simulink library "Lib_Piccolo"  (R2018b)
settings: Solver=VariableStepAuto  StartTime=0.0  StopTime=10.0  RelTol=1e-3
values from neighbouring files (symbols this model uses):
  AccelErrInt2Brakes = 0.15    [SimulationControlConfig16P.m]    (also in SimulationControlConfig16P_LEGACY.m; SimulationControlConfigTAILLESS.m = 0.2; SimulationControlConfigUTAIL.m = 0.2)
  AileronMax = 25    [SimulationControlConfig16P.m]    (also in SimulationControlConfig16P_LEGACY.m; SimulationControlConfigTAILLESS.m; SimulationControlConfigUTAIL.m)
  AileronPower = 0.00268    [SimulationControlConfig16P.m]    (also in SimulationControlConfig16P_LEGACY.m; SimulationControlConfigTAILLESS.m; SimulationControlConfigUTAIL.m)
  AileronSurfaceMax = 45    [SimulationControlConfig16P.m]    (also in SimulationControlConfig16P_LEGACY.m)
  AileronTrim = 0    [SimulationControlConfig16P.m]    (also in SimulationControlConfig16P_LEGACY.m; SimulationControlConfigTAILLESS.m; SimulationControlConfigUTAIL.m)
  Alt = 1000 + TerrainHeight    [SimulationStateConfig.m]
  AltCruise_m = testPlans(testIndx).terrainElevation * 0.3048 + 200    [SimulationControlConfig16P.m]    (also in SimulationControlConfigTAILLESS.m = 1083; SimulationControlConfigUTAIL.m = testPlans(testIndx).terrainElevation * 0.3048 + 152)
  AltitudeRate2PitchCmdIntegratorInit = 0.1    [SimulationControlPre.m]
  AltMax = 10000    [SimulationControlConfig16P.m]    (also in SimulationControlConfig16P_LEGACY.m; SimulationControlConfigTAILLESS.m; SimulationControlConfigUTAIL.m)
  AltMaxAccel = 1.25    [SimulationControlConfig16P.m]    (also in SimulationControlConfig16P_LEGACY.m = 0.9; SimulationControlConfigTAILLESS.m = 1.7; SimulationControlConfigUTAIL.m = 2)
  AltMin = 0    [SimulationControlConfig16P.m]    (also in SimulationControlConfig16P_LEGACY.m; SimulationControlConfigTAILLESS.m; SimulationControlConfigUTAIL.m)
  AltRateCmd2Pitch = 0.50    (= 0.5)    [SimulationControlConfig16P.m]    (also in SimulationControlConfig16P_LEGACY.m = 0.6; SimulationControlConfigTAILLESS.m = 0.2; SimulationControlConfigUTAIL.m = 0.3)
  AltRateError2Pitch = 0.40    (= 0.4)    [SimulationControlConfig16P.m]    (also in SimulationControlConfig16P_LEGACY.m; SimulationControlConfigTAILLESS.m = 0.55; SimulationControlConfigUTAIL.m = 0.55)
  AltRateErrorInt2Pitch = 0.50    (= 0.5)    [SimulationControlConfig16P.m]    (also in SimulationControlConfig16P_LEGACY.m = 0.45; SimulationControlConfigTAILLESS.m; SimulationControlConfigUTAIL.m = 0.75)
  AltRateLpfCutOff = 3    [SimulationControlConfig16P.m]    (also in SimulationControlConfig16P_LEGACY.m; SimulationControlConfigTAILLESS.m = 2; SimulationControlConfigUTAIL.m = 2)
  AutoNosegear2Rudder = 26    [SimulationControlConfig16P.m]    (also in SimulationControlConfig16P_LEGACY.m; SimulationControlConfigTAILLESS.m = 25.2; SimulationControlConfigUTAIL.m = 14)
  b = 5.54    [SimulationControlConfig16P.m]    (also in SimulationControlConfig16P_LEGACY.m; SimulationControlConfigTAILLESS.m = 2.37; SimulationControlConfigUTAIL.m = 2.37)
  Bank2AileronIntegratorInit = 0    [SimulationControlPre.m]
  BankMax_User = BankMax_User/180*pi    (= 0.523598775598)    [SimulationControlConfig16P.m]    (also in SimulationControlConfig16P_LEGACY.m; SimulationControlConfigTAILLESS.m = 0.610865238198; SimulationControlConfigUTAIL.m = 0.628318530718)
  baseLegFlaps = 20    [SimulationControlConfig16P.m]    (also in SimulationControlConfig16P_LEGACY.m = 0; SimulationControlConfigTAILLESS.m = 15; SimulationControlConfigUTAIL.m = 10)
  C = GeneticOpt.C    [SimulationCostFunction.m]
  c = Sw/b    (= 0.841696750903)    [SimulationControlConfig16P.m]    (also in SimulationControlConfig16P_LEGACY.m; SimulationControlConfigTAILLESS.m = 0.354008438819; SimulationControlConfigUTAIL.m = 0.354008438819)
  cell2WheelFactorMG = 5.98    [SimulationSensorConfig16P_LEGACY.m]
  cell2WheelFactorNG = 1    [SimulationSensorConfig16P_LEGACY.m]
  cellSatMaxMG = 15000    [SimulationSensorConfig16P.m]    (also in SimulationSensorConfig16P_LEGACY.m; SimulationSensorConfigTAILLESS7P.m; SimulationSensorConfigUTAIL7P.m)
  cellSatMaxNG = 1000    [SimulationSensorConfig16P.m]    (also in SimulationSensorConfig16P_LEGACY.m; SimulationSensorConfigTAILLESS7P.m; SimulationSensorConfigUTAIL7P.m)
  cellSatMinMG = -15000    [SimulationSensorConfig16P.m]    (also in SimulationSensorConfig16P_LEGACY.m; SimulationSensorConfigTAILLESS7P.m; SimulationSensorConfigUTAIL7P.m)
  cellSatMinNG = -1000    [SimulationSensorConfig16P.m]    (also in SimulationSensorConfig16P_LEGACY.m; SimulationSensorConfigTAILLESS7P.m; SimulationSensorConfigUTAIL7P.m)
  CL_Limit = CL_Max    (= 0.54)    [SimulationControlConfig16P.m]    (also in SimulationControlConfig16P_LEGACY.m; SimulationControlConfigTAILLESS.m; SimulationControlConfigUTAIL.m = 0.53)
  CL_Max = 0.54    [SimulationControlConfig16P.m]    (also in SimulationControlConfig16P_LEGACY.m; SimulationControlConfigTAILLESS.m; SimulationControlConfigUTAIL.m = 0.53)
  CL_Max_Nom = 0.465    [SimulationControlConfig16P.m]    (also in SimulationControlConfig16P_LEGACY.m; SimulationControlConfigTAILLESS.m = 0.39; SimulationControlConfigUTAIL.m)
  CL_Min = 0    [SimulationControlConfig16P.m]    (also in SimulationControlConfig16P_LEGACY.m; SimulationControlConfigTAILLESS.m; SimulationControlConfigUTAIL.m)
  ClimbMaxFraction = 0.35    [SimulationControlConfig16P.m]    (also in SimulationControlConfig16P_LEGACY.m = 0.24; SimulationControlConfigTAILLESS.m = 0.19; SimulationControlConfigUTAIL.m = 0.21)
  ClimboutMaxBank = 7.0    (= 7)    [SimulationControlConfig16P.m]    (also in SimulationControlConfig16P_LEGACY.m; SimulationControlConfigTAILLESS.m = 5; SimulationControlConfigUTAIL.m)
  ClimboutTimer = 7.0    (= 7)    [SimulationControlConfig16P.m]    (also in SimulationControlConfig16P_LEGACY.m; SimulationControlConfigTAILLESS.m; SimulationControlConfigUTAIL.m)
  dCl_per_dFlap = 0.005581818    [SimulationControlConfig16P.m]    (also in SimulationControlConfig16P_LEGACY.m = 0; SimulationControlConfigTAILLESS.m = 0; SimulationControlConfigUTAIL.m = 0)
  DecelerationCmd = 3.1    [SimulationControlConfig16P.m]    (also in SimulationControlConfig16P_LEGACY.m; SimulationControlConfigTAILLESS.m = 0.1; SimulationControlConfigUTAIL.m = 0.1)
  DeRotateLogicEndTimer = abs((NoseDownLimit_Deg-1)/DeRotateRamp_Dps)    [SimulationControlConfig16P.m]    (also in SimulationControlConfig16P_LEGACY.m; SimulationControlConfigTAILLESS.m; SimulationControlConfigUTAIL.m)
  DeRotateLogicHoldNoseUpTimer = 0.1    [SimulationControlConfig16P.m]    (also in SimulationControlConfig16P_LEGACY.m; SimulationControlConfigTAILLESS.m; SimulationControlConfigUTAIL.m)
  DeRotateLogicTimerTimeout = 2    [SimulationControlConfig16P.m]    (also in SimulationControlConfig16P_LEGACY.m; SimulationControlConfigTAILLESS.m; SimulationControlConfigUTAIL.m)
  DeRotateLowerCmdSaturation = 0    [SimulationControlConfig16P.m]    (also in SimulationControlConfig16P_LEGACY.m; SimulationControlConfigTAILLESS.m; SimulationControlConfigUTAIL.m)
  DeRotateRamp_Dps = 3    [SimulationControlConfig16P.m]    (also in SimulationControlConfig16P_LEGACY.m; SimulationControlConfigTAILLESS.m = 8; SimulationControlConfigUTAIL.m = 8)
  DeRotateUpperCmdSaturation = 7    [SimulationControlConfig16P.m]    (also in SimulationControlConfig16P_LEGACY.m; SimulationControlConfigTAILLESS.m; SimulationControlConfigUTAIL.m)
  DescentMaxFraction = 0.22    [SimulationControlConfig16P.m]    (also in SimulationControlConfig16P_LEGACY.m = 0.2; SimulationControlConfigTAILLESS.m = 0.17; SimulationControlConfigUTAIL.m = 0.17)
  DesktopSimTerrainOffset_m = 0.406    [SimulationAircraftConfig.m]
  downwindFlaps = 0    [SimulationControlConfig16P.m]    (also in SimulationControlConfig16P_LEGACY.m; SimulationControlConfigTAILLESS.m; SimulationControlConfigUTAIL.m)
  DP_init = 0.5*1.225*V_init^2    [SimulationControlConfig16P.m]    (also in SimulationControlConfig16P_LEGACY.m; SimulationControlConfigTAILLESS.m; SimulationControlConfigUTAIL.m)
  dscNoiseMG = 1    [SimulationSensorConfig16P_LEGACY.m]
  dscNoiseNG = 0.25    [SimulationSensorConfig16P_LEGACY.m]
  DSCnumBits = 24    [SimulationSensorConfig16P.m]    (also in SimulationSensorConfig16P_LEGACY.m; SimulationSensorConfigTAILLESS7P.m; SimulationSensorConfigUTAIL7P.m)
  DSCRangeMaxMG = 15000    [SimulationSensorConfig16P.m]    (also in SimulationSensorConfig16P_LEGACY.m; SimulationSensorConfigTAILLESS7P.m; SimulationSensorConfigUTAIL7P.m)
  DSCRangeMaxNG = 1000    [SimulationSensorConfig16P.m]    (also in SimulationSensorConfig16P_LEGACY.m; SimulationSensorConfigTAILLESS7P.m; SimulationSensorConfigUTAIL7P.m)
  DSCRangeMinMG = -15000    [SimulationSensorConfig16P.m]    (also in SimulationSensorConfig16P_LEGACY.m; SimulationSensorConfigTAILLESS7P.m; SimulationSensorConfigUTAIL7P.m)
  DSCRangeMinNG = -1000    [SimulationSensorConfig16P.m]    (also in SimulationSensorConfig16P_LEGACY.m; SimulationSensorConfigTAILLESS7P.m; SimulationSensorConfigUTAIL7P.m)
  dt = DLLSim.dt    [SimulationTimeStep.m]    (also in SimulationTrim.m = 0.02)
  EarlyTouchdownThreshold = 3.0    (= 3)    [SimulationControlConfig16P.m]    (also in SimulationControlConfig16P_LEGACY.m; SimulationControlConfigTAILLESS.m = 2.2; SimulationControlConfigUTAIL.m = 2.5)
  ElevatorDeflectionRate = 15    [SimulationControlConfig16P.m]    (also in SimulationControlConfig16P_LEGACY.m = 12; SimulationControlConfigTAILLESS.m = 10; SimulationControlConfigUTAIL.m = 12)
  ElevatorMax = 25    [SimulationControlConfig16P.m]    (also in SimulationControlConfig16P_LEGACY.m; SimulationControlConfigTAILLESS.m; SimulationControlConfigUTAIL.m)
  ElevatorPower = -0.002209    [SimulationControlConfig16P.m]    (also in SimulationControlConfig16P_LEGACY.m; SimulationControlConfigTAILLESS.m = -0.002956; SimulationControlConfigUTAIL.m = -0.00205983)
  ElevatorTrim = -3.5    [SimulationControlConfig16P.m]    (also in SimulationControlConfig16P_LEGACY.m; SimulationControlConfigTAILLESS.m = -6; SimulationControlConfigUTAIL.m = -8)
  elevonBias = 0    [SimulationControlConfig16P.m]    (also in SimulationControlConfig16P_LEGACY.m; SimulationControlConfigTAILLESS.m; SimulationControlConfigUTAIL.m)
  Enable_TAS_Protection = 0    [SimulationControlConfig16P.m]    (also in SimulationControlConfig16P_LEGACY.m; SimulationControlConfigTAILLESS.m; SimulationControlConfigUTAIL.m)
  EnableCrossTrackAbort = 1    [SimulationControlConfig16P.m]    (also in SimulationControlConfigTAILLESS.m; SimulationControlConfigUTAIL.m)
  EnergyBandwidth = 0.02    [SimulationControlConfig16P.m]    (also in SimulationControlConfig16P_LEGACY.m; SimulationControlConfigTAILLESS.m = 0.06; SimulationControlConfigUTAIL.m = 0.06)
  EngineLhFuelCut = 0    [SimulationAircraftConfig.m]
  EngineRhFuelCut = 0    [SimulationAircraftConfig.m]
  FastThrottleRate = 0.075    [SimulationControlConfig16P.m]    (also in SimulationControlConfig16P_LEGACY.m = 0.05; SimulationControlConfigTAILLESS.m = 0.1; SimulationControlConfigUTAIL.m = 0.1)
  FilterWarmUpTime = 2    [SimulationSensorConfig16P.m]    (also in SimulationSensorConfig16P_LEGACY.m; SimulationSensorConfigTAILLESS7P.m; SimulationSensorConfigUTAIL7P.m)
  finalApproachFlaps = 20    [SimulationControlConfig16P.m]    (also in SimulationControlConfig16P_LEGACY.m = 0; SimulationControlConfigTAILLESS.m = 22; SimulationControlConfigUTAIL.m = 10)
  FinalDescentSlope_Deg = testPlans(testIndx).descentSlope    [SimulationControlConfig16P.m]    (also in SimulationControlConfig16P_LEGACY.m; SimulationControlConfigTAILLESS.m; SimulationControlConfigUTAIL.m)
  flapMax = 0    [SimulationControlConfig16P.m]    (also in SimulationControlConfig16P_LEGACY.m; SimulationControlConfigTAILLESS.m; SimulationControlConfigUTAIL.m)
  flapRate = 7.5    [SimulationControlConfig16P.m]    (also in SimulationControlConfig16P_LEGACY.m; SimulationControlConfigTAILLESS.m = 6.6; SimulationControlConfigUTAIL.m)
  FlareHeight = 5    [SimulationControlConfig16P.m]    (also in SimulationControlConfig16P_LEGACY.m = 4.8; SimulationControlConfigTAILLESS.m = 2.5; SimulationControlConfigUTAIL.m = 2)
  FlareVerticalRate_mps = -0.4    [SimulationControlConfig16P.m]    (also in SimulationControlConfig16P_LEGACY.m = -0.5; SimulationControlConfigTAILLESS.m = -0.15; SimulationControlConfigUTAIL.m = -0.15)
  Fp_Aileron = 0.55*2*pi*RollRateLpfCutoff*dt    [SimulationControlConfig16P.m]    (also in SimulationControlConfig16P_LEGACY.m; SimulationControlConfigTAILLESS.m; SimulationControlConfigUTAIL.m)
  Fp_Alt = 0.55*AltBandwidth    (= 0.099)    [SimulationControlConfig16P.m]    (also in SimulationControlConfig16P_LEGACY.m; SimulationControlConfigTAILLESS.m = 0.587477826221; SimulationControlConfigUTAIL.m = 0.69115038379)
  Fp_AltRate = 0.55*2*pi*AltRateLpfCutOff*dt    [SimulationControlConfig16P.m]    (also in SimulationControlConfig16P_LEGACY.m; SimulationControlConfigTAILLESS.m; SimulationControlConfigUTAIL.m)
  Fp_Elevator = 0.55*2*pi*PitchRateLpfCutoff*dt    [SimulationControlConfig16P.m]    (also in SimulationControlConfig16P_LEGACY.m; SimulationControlConfigTAILLESS.m; SimulationControlConfigUTAIL.m)
  Fp_Energy = 0.55*2*pi*EnergyBandwidth    (= 0.069115038379)    [SimulationControlConfig16P.m]    (also in SimulationControlConfig16P_LEGACY.m; SimulationControlConfigTAILLESS.m = 0.207345115137; SimulationControlConfigUTAIL.m = 0.207345115137)
  Fp_Energy2 = 0.55*2*pi*EnergyBandwidth*dt    [SimulationControlConfig16P.m]    (also in SimulationControlConfig16P_LEGACY.m; SimulationControlConfigTAILLESS.m; SimulationControlConfigUTAIL.m)
  Fp_Pitch = 0.55*2*pi*PitchBandwidth    (= 2.76460153516)    [SimulationControlConfig16P.m]    (also in SimulationControlConfig16P_LEGACY.m = 3.11017672705; SimulationControlConfigTAILLESS.m = 3.80132711084; SimulationControlConfigUTAIL.m = 2.41902634326)
  Fp_Pitch_2 = 0.55*2*pi*PitchBandwidth*dt    [SimulationControlConfig16P.m]    (also in SimulationControlConfig16P_LEGACY.m; SimulationControlConfigTAILLESS.m; SimulationControlConfigUTAIL.m)
  Fp_Roll = RollBandwidth^2    (= 1)    [SimulationControlConfig16P.m]    (also in SimulationControlConfig16P_LEGACY.m = 1.44; SimulationControlConfigTAILLESS.m; SimulationControlConfigUTAIL.m)
  Fp_Rudder = 0.55*2*pi*YawRateLpfCutoff*dt    [SimulationControlConfig16P.m]    (also in SimulationControlConfig16P_LEGACY.m; SimulationControlConfigTAILLESS.m; SimulationControlConfigUTAIL.m)
  Fp_TAS = 0.55*2*pi*TASBandwidth    (= 0.103672557568)    [SimulationControlConfig16P.m]    (also in SimulationControlConfig16P_LEGACY.m; SimulationControlConfigTAILLESS.m = 0.172787595947; SimulationControlConfigUTAIL.m = 0.172787595947)
  Fp_TAS_Filter = 2*pi*TasLpfCutoff*dt    [SimulationControlConfig16P.m]    (also in SimulationControlConfig16P_LEGACY.m; SimulationControlConfigTAILLESS.m; SimulationControlConfigUTAIL.m)
  Fp_Turn = 0.55*2*pi*TurnErrLPFcutoff    (= 0.0345575191895)    [SimulationControlConfig16P.m]    (also in SimulationControlConfig16P_LEGACY.m; SimulationControlConfigTAILLESS.m = 0.172787595947; SimulationControlConfigUTAIL.m = 0.172787595947)
  Fp_TurnDerr = 0.55*2*pi*TurnDerivativeLPFcutoff    (= 0.0345575191895)    [SimulationControlConfig16P.m]    (also in SimulationControlConfig16P_LEGACY.m; SimulationControlConfigTAILLESS.m = 0.172787595947; SimulationControlConfigUTAIL.m = 0.172787595947)
  FTV = 3    [SimulationAircraftConfig.m]
  ftvStaticPositionError = 1/1.18    (= 0.847457627119)    [SimulationSensorConfig16P.m]    (also in SimulationSensorConfig16P_LEGACY.m; SimulationSensorConfigTAILLESS7P.m = 1; SimulationSensorConfigUTAIL7P.m = 1)
  g = 9.81    [SimulationStateConfig.m]
  GustSpd_Kts = testPlans(testIndx).gustSpd    [SimulationStateConfig.m]
  GustTriggerVal = testPlans(testIndx).gustTriggerVal    [SimulationStateConfig.m]
  HeadingErr2TurnRate = 0.5    [SimulationControlConfig16P.m]    (also in SimulationControlConfig16P_LEGACY.m; SimulationControlConfigTAILLESS.m; SimulationControlConfigUTAIL.m)
  HeadingErrDer2TurnRate = 0.3    [SimulationControlConfig16P.m]    (also in SimulationControlConfig16P_LEGACY.m; SimulationControlConfigTAILLESS.m; SimulationControlConfigUTAIL.m)
  IASbounce = IASstall*0.8    [SimulationControlPre.m]
  IAScruiseCMD = sqrt(2*m*9.81/(1.225*Sw*CL_cruise))    [SimulationControlConfig16P.m]    (also in SimulationControlConfig16P_LEGACY.m; SimulationControlConfigTAILLESS.m; SimulationControlConfigUTAIL.m)
  IASfinalCMD = 1.12 * IASmin    [SimulationControlConfig16P.m]    (also in SimulationControlConfig16P_LEGACY.m = 1.10 * IASmin; SimulationControlConfigTAILLESS.m = 1.10 * IASmin; SimulationControlConfigUTAIL.m = 1.15 * IASmin)
  IASflareCMD = IASstall    [SimulationControlConfig16P.m]    (also in SimulationControlConfig16P_LEGACY.m; SimulationControlConfigTAILLESS.m; SimulationControlConfigUTAIL.m)
  IASmax = 64    [SimulationControlConfig16P.m]    (also in SimulationControlConfig16P_LEGACY.m = 46; SimulationControlConfigTAILLESS.m = 38.58; SimulationControlConfigUTAIL.m = 35)
  IASmin = sqrt(2*m*9.81/(1.225*Sw*0.9*CL_Max_Nom))    [SimulationControlConfig16P.m]    (also in SimulationControlConfig16P_LEGACY.m; SimulationControlConfigTAILLESS.m; SimulationControlConfigUTAIL.m)
  IASshortCMD = IASstall    [SimulationControlConfig16P.m]    (also in SimulationControlConfig16P_LEGACY.m; SimulationControlConfigTAILLESS.m; SimulationControlConfigUTAIL.m)
  IASstall = sqrt(2*m*9.81/(1.225*Sw*CL_Max))    [SimulationControlConfig16P.m]    (also in SimulationControlConfig16P_LEGACY.m; SimulationControlConfigTAILLESS.m; SimulationControlConfigUTAIL.m)
  inFlight = 1    [SimulationControlConfig16P.m]    (also in SimulationControlConfigTAILLESS.m; SimulationControlConfigUTAIL.m)
  JetCatOffset = 5    [SimulationControlConfig16P.m]    (also in SimulationControlConfig16P_LEGACY.m)
  LaunchRollingElevator = -1.5    [SimulationControlConfig16P.m]    (also in SimulationControlConfig16P_LEGACY.m; SimulationControlConfigTAILLESS.m = 1; SimulationControlConfigUTAIL.m = 1)
  ldg_NosegearMax = 10    [SimulationControlConfig16P.m]    (also in SimulationControlConfig16P_LEGACY.m; SimulationControlConfigTAILLESS.m; SimulationControlConfigUTAIL.m)
  ldg_TrackVyErrInt2Nosegear = 0.1250    (= 0.125)    [SimulationControlConfig16P.m]    (also in SimulationControlConfig16P_LEGACY.m; SimulationControlConfigTAILLESS.m = 0.00714285714286; SimulationControlConfigUTAIL.m = 0.00714285714286)
  ldg_TrackVyErrPro2Nosegear = 0.35    [SimulationControlConfig16P.m]    (also in SimulationControlConfig16P_LEGACY.m; SimulationControlConfigTAILLESS.m = 0.0546666666667; SimulationControlConfigUTAIL.m = 0.0546666666667)
  ldg_TrackY2Vy = 0.07    [SimulationControlConfig16P.m]    (also in SimulationControlConfig16P_LEGACY.m; SimulationControlConfigTAILLESS.m = 0.17; SimulationControlConfigUTAIL.m = 0.17)
  ldg_Vy2NosegearScalingPower = 1.075    [SimulationControlConfig16P.m]    (also in SimulationControlConfig16P_LEGACY.m; SimulationControlConfigTAILLESS.m = 0.6; SimulationControlConfigUTAIL.m = 0.5)
  ldg_Y2VyScalingPower = 0.175    [SimulationControlConfig16P.m]    (also in SimulationControlConfig16P_LEGACY.m; SimulationControlConfigTAILLESS.m = 0; SimulationControlConfigUTAIL.m = 0)
  ldg_YawRate2Nosegear = 0.175    [SimulationControlConfig16P.m]    (also in SimulationControlConfig16P_LEGACY.m; SimulationControlConfigTAILLESS.m = 0.065; SimulationControlConfigUTAIL.m = 0.065)
  LiftSlope = 0.064285    [SimulationControlConfig16P.m]    (also in SimulationControlConfig16P_LEGACY.m; SimulationControlConfigTAILLESS.m = 0.058631; SimulationControlConfigUTAIL.m)
  LPFaileronInit = 0    [SimulationControlPre.m]
  LPFclestInit = 0    [SimulationControlPre.m]
  LPFenergyFFInit = 0    [SimulationControlPre.m]
  LPFtasInit = V_init + 2    [SimulationControlPre.m]
  LPFthrottleInit = ThrottleTrim    [SimulationControlPre.m]
  LPFturnErrInit = 0    [SimulationControlPre.m]
  ... (+115 more)
undefined symbols (not defined in the file or in its folder): abortFlag, alphaHPF, apmDelay, BRWNOUT, CRAWOR, CRAWUR, DiscIntNeverNeededParam, DLLSim, DLLSimStep, ECOMOR, ECOMUR, Fp_Tas, GustTrigger_HeightAgl_m, IPSTAT, LCINTEG, Ldg_Persist_Time, LOWER_FLAGS, MSG_ENABLE, NoiseStd, OLDVAL, OVERRIDE_ENABLE, OVERRIDE_VALUE, REBOOT, reversionEnable, revIASMax, revIASMin, revPitchMax, revPitchMin, revPitchRateMax, revRollMax, revRollRateMax, SAMPLE, SCALON, SensorModel, sigbuilder_block, Sim_Vx, Sim_Vy, Sim_Vz, Sim_Xpos, Sim_Ypos, Sim_Zpos, SYSOR, SYSUR, TARE, TEMPOR, TEMPUR, testIndx, testPlan, testPlans, Trim_piccoloInCmd, Trim_REFSI_FD_IN_nmodeCgShifterCmd_Ft, Trim_REFSI_FD_IN_nmodeFlapLhIBCmd_Deg, Trim_REFSI_FD_IN_nmodeFlapLhOBCmd_Deg, Trim_REFSI_FD_IN_nmodeFlapRhIBCmd_Deg, Trim_REFSI_FD_IN_nmodeFlapRhOBCmd_Deg, Trim_REFSI_FD_IN_nmodeSlatLhCmd_Deg, Trim_REFSI_FD_IN_nmodeSlatRhCmd_Deg, Trim_REFSI_FD_IN_nmodeSplrLhInbdCmd_Deg, Trim_REFSI_FD_IN_nmodeSplrLhOutbdCmd_Deg ... (+5)
libraries: simulink x866, aerolibconvert2 x60, $bdroot x52, aerolibatmos2 x5, dspswit3 x5, simulink_extras x4, dsparch4 x2, Lib_Piccolo_Alt x2, eeGeneralControl x1, dspindex x1
(part 5 of 44)

== system Lib_Piccolo/Steering Controller Landing ==
  Y command : Inport
  Feedback : Inport  Port=2
  Bus Selector : BusSelector  OutputSignals=Sim_VGround,Sim_Ypos,Sim_Vy,YawRate_Body_radps
  Constant : Constant  Value=0
  Constant1 : Constant  Value=0
  Gain3 : Gain  Gain=1/4
  Gain4 : Gain  Gain=-1
  Integrator1 : Integrator  ExternalReset=level
  NOT : Logic  Operator=NOT  IconShape=distinctive  AllPortsSameDT=off  OutDataTypeStr=boolean
  "Nosegear rudder mixer " : Subsystem
  Nosegear scaling based on ground speed : Subsystem
  Product2 : Product
  Product3 : Product
  Saturation Dynamic1 : simulink/Discontinuities/Saturation Dynamic  OutMin=[]  OutMax=[]  OutDataTypeStr=Inherit: Same as second input  OutDataType=fixdt(1, 16)  OutScaling=2^-10  DoSatur=off
  Sum4 : Sum  Inputs=|++
  Sum5 : Sum  Inputs=|+-
  Sum6 : Sum  Inputs=+-|
  Sum7 : Sum  Inputs=|+-
  Switch : Switch  Criteria=u2 > Threshold  Threshold=1.5
  Switch1 : Switch  Criteria=u2 > Threshold  Threshold=1.5
  "Track Vy error integral to nosegear " : Gain  Gain=ldg_TrackVyErrInt2Nosegear
  "Track Vy error to nosegear " : Gain  Gain=ldg_TrackVyErrPro2Nosegear
  Track Y to Vy : Gain  Gain=ldg_TrackY2Vy
  Vy scaling based on ground speed : Subsystem
  Vy to nosegear scaling power : Constant  Value=ldg_Vy2NosegearScalingPower
  "Y to Vy scaling power " : Constant  Value=ldg_Y2VyScalingPower
  Yaw rate to nosegear : Gain  Gain=ldg_YawRate2Nosegear
  Rudder_Deg : Outport
  Nosegear_Deg : Outport  Port=2
  wires:
  Y command/1 -> Sum6/1  "Sim.YCmd"
  Feedback/1 -> Bus Selector/1
  "Nosegear rudder mixer "/1(Nosegear command) -> Nosegear_Deg/1  "Sim.NosegearCmd"
  "Y to Vy scaling power "/1 -> Vy scaling based on ground speed/2(Y to Vy scaling power)
  Product2/1 -> Saturation Dynamic1/2
  Gain3/1 -> Saturation Dynamic1/1, Gain4/1
  Constant/1 -> Switch/3
  "Track Vy error integral to nosegear "/1 -> Sum4/2  "Ki_Vy"
  Yaw rate to nosegear/1 -> Sum5/2  "Sim.YawRate2Nosegear"
  "Track Vy error to nosegear "/1 -> Sum4/1  "Kp_Vy"
  Switch1/1 -> Gain3/1
  Switch/1 -> "Nosegear rudder mixer "/1("Desired nosegear ")
  Sum5/1 -> Switch/1
  Saturation Dynamic1/1 -> Sum7/1  "Sim.VyCmd"
  Nosegear scaling based on ground speed/1(nosegear scalar) -> Product3/1  "Sim.NosegearScalar"
  Bus Selector/1 -> Nosegear scaling based on ground speed/1(Ground Speed), Switch/2, Vy scaling based on ground speed/1(Ground Speed), Switch1/2, Switch1/1  "<Sim_VGround>"
  Vy scaling based on ground speed/1(Vy Scalar) -> Product2/1  "Sim.Vy Scalar"
  Constant1/1 -> Switch1/3
  Vy to nosegear scaling power/1 -> Nosegear scaling based on ground speed/2("Vy to nosegear scaling ")
  Gain4/1 -> Saturation Dynamic1/3
  Integrator1/1 -> "Track Vy error integral to nosegear "/1
  Track Y to Vy/1 -> Product2/2
  Sum4/1 -> Product3/2
  Bus Selector/3 -> Sum7/2  "<Sim_Vy>"
  Bus Selector/2 -> Sum6/2  "<Sim_Ypos>"
  Product3/1 -> Sum5/1
  "Nosegear rudder mixer "/2(Rudder command) -> Rudder_Deg/1  "Sim.RudderCmd"
  Sum6/1 -> Track Y to Vy/1  "TrackY Error"
  Sum7/1 -> "Track Vy error to nosegear "/1, Integrator1/1  "Sim.Vy Error"
  Bus Selector/4 -> Yaw rate to nosegear/1  "<YawRate_Body_radps>"
  [Rollout_Flag] -> NOT/1
  NOT/1 -> Integrator1/2

== system Lib_Piccolo/Steering Controller Selection ==
  Rollout Rudder In : Inport
  Rollout NG In : Inport  Port=2
  Transition Rudder In : Inport  Port=3
  Transition NG In : Inport  Port=4
  Switch : Switch  Threshold=5
  Switch1 : Switch  Threshold=5
  Rudder_Deg : Outport
  Nosegear_Deg : Outport  Port=2
  wires:
  [Pic_AP_Mode] -> Switch1/2, Switch/2
  Rollout Rudder In/1 -> Switch/1  "Rollout_Rud"
  Transition Rudder In/1 -> Switch/3  "Transition_Rud"
  Switch/1 -> Rudder_Deg/1
  Switch1/1 -> Nosegear_Deg/1
  Rollout NG In/1 -> Switch1/1  "Rollout_NG"
  Transition NG In/1 -> Switch1/3  "Transition_NG"

== system Lib_Piccolo/Steering Controller Transition ==
  Y command : Inport
  Feedback : Inport  Port=2
  AND : Logic  IconShape=distinctive  AllPortsSameDT=off  OutDataTypeStr=boolean
  Abs : Abs
  Bus Selector : BusSelector  OutputSignals=Sim_VGround,Sim_Ypos,Sim_Vy,YawRate_Body_radps
  Compare To Constant : simulink/Logic and Bit Operations/Compare To Constant  relop=>=  const=MaxCrossError  OutDataTypeStr=boolean
  Compare To Constant1 : simulink/Logic and Bit Operations/Compare To Constant  relop===  const=1  OutDataTypeStr=boolean
  Constant : Constant  Value=0
  Constant1 : Constant  Value=0
  Gain3 : Gain  Gain=1/4
  Gain4 : Gain  Gain=-1
  Integrator1 : Integrator  ExternalReset=level
  "Nosegear rudder mixer " : Subsystem
  Nosegear scaling based on ground speed : Subsystem
  Product2 : Product
  Product3 : Product
  Saturation Dynamic1 : simulink/Discontinuities/Saturation Dynamic  OutMin=[]  OutMax=[]  OutDataTypeStr=Inherit: Same as second input  OutDataType=fixdt(1, 16)  OutScaling=2^-10  DoSatur=off
  Sum4 : Sum  Inputs=|++
  Sum5 : Sum  Inputs=|+-
  Sum6 : Sum  Inputs=+-|
  Sum7 : Sum  Inputs=|+-
  Switch : Switch  Criteria=u2 > Threshold  Threshold=1.5
  Switch1 : Switch  Criteria=u2 > Threshold  Threshold=1.5
  "Track Vy error integral to nosegear " : Gain  Gain=TrackVyErrInt2Nosegear
  "Track Vy error to nosegear " : Gain  Gain=TrackVyErrPro2Nosegear
  Track Y to Vy : Gain  Gain=TrackY2Vy
  Vy scaling based on ground speed : Subsystem
  Vy to nosegear scaling power : Constant  Value=Vy2NosegearScalingPower
  "Y to Vy scaling power " : Constant  Value=Y2VyScalingPower
  Yaw rate to nosegear : Gain  Gain=YawRate2Nosegear
  Rudder_Deg : Outport
  Nosegear_Deg : Outport  Port=2
  tag scope: Flag_CrossTrackAbort=global
  wires:
  Y command/1 -> Sum6/1  "Sim.YCmd"
  Feedback/1 -> Bus Selector/1
  "Nosegear rudder mixer "/1(Nosegear command) -> Nosegear_Deg/1  "Sim.NosegearCmd"
  "Y to Vy scaling power "/1 -> Vy scaling based on ground speed/2(Y to Vy scaling power)
  Product2/1 -> Saturation Dynamic1/2
  Gain3/1 -> Saturation Dynamic1/1, Gain4/1
  Constant/1 -> Switch/3
  "Track Vy error integral to nosegear "/1 -> Sum4/2  "Ki_Vy"
  Yaw rate to nosegear/1 -> Sum5/2  "Sim.YawRate2Nosegear"
  "Track Vy error to nosegear "/1 -> Sum4/1  "Kp_Vy"
  Switch1/1 -> Gain3/1
  Switch/1 -> "Nosegear rudder mixer "/1("Desired nosegear ")
  Sum5/1 -> Switch/1
  Saturation Dynamic1/1 -> Sum7/1  "Sim.VyCmd"
  Nosegear scaling based on ground speed/1(nosegear scalar) -> Product3/1  "Sim.NosegearScalar"
  Bus Selector/1 -> Switch/2, Nosegear scaling based on ground speed/1(Ground Speed), Vy scaling based on ground speed/1(Ground Speed), Switch1/2, Switch1/1  "<Sim_VGround>"
  Vy scaling based on ground speed/1(Vy Scalar) -> Product2/1  "Sim.Vy Scalar"
  Constant1/1 -> Switch1/3
  Vy to nosegear scaling power/1 -> Nosegear scaling based on ground speed/2("Vy to nosegear scaling ")
  Gain4/1 -> Saturation Dynamic1/3
  Integrator1/1 -> "Track Vy error integral to nosegear "/1
  Track Y to Vy/1 -> Product2/2
  Sum4/1 -> Product3/2
  Bus Selector/3 -> Sum7/2  "<Sim_Vy>"
  Bus Selector/2 -> Sum6/2  "<Sim_Ypos>"
  Product3/1 -> Sum5/1
  "Nosegear rudder mixer "/2(Rudder command) -> Rudder_Deg/1  "Sim.RudderCmd"
  Sum6/1 -> Abs/1, Track Y to Vy/1  "TrackY Error"
  Sum7/1 -> "Track Vy error to nosegear "/1, Integrator1/1  "Sim.Vy Error"
  Bus Selector/4 -> Yaw rate to nosegear/1  "<YawRate_Body_radps>"
  [Rollout_Flag] -> Integrator1/2
  Abs/1 -> Compare To Constant/1
  Compare To Constant/1 -> AND/2
  [Pic_AP_Mode] -> Compare To Constant1/1
  AND/1 -> [Flag_CrossTrackAbort]  "Flag_CrossTrackAbort"
  Compare To Constant1/1 -> AND/1

== system Lib_Piccolo/TLA Selection ==
  Airspeed_TLA : Inport
  Alt_TLA : Inport  Port=2
  Rate Limiter : RateLimiter  RisingSlewLimit=ThrottleRateMax  FallingSlewLimit=-ThrottleRateMax  SampleTimeMode=inherited
  Switch4 : Switch  Criteria=u2 > Threshold
  Sim_ThrottleCmd : Outport
  wires:
  [Flag_TAS_Priority] -> Switch4/2
  Alt_TLA/1 -> Switch4/3
  Airspeed_TLA/1 -> Switch4/1
  Switch4/1 -> Rate Limiter/1
  Rate Limiter/1 -> Sim_ThrottleCmd/1

== system Lib_Piccolo/Throttle Control (Airspeed Mode) ==
  hCmd : Inport
  Vcmd : Inport  Port=2
  Feedback Bus : Inport  Port=3
  " " : Constant  Value=ThrottleTrim
  " TLASaturation 1" : Saturate  UpperLimit=ThrottleMax  LowerLimit=ThrottleMin  LinearizeAsGain=off
  "1/ MaxEnginePower " : Gain  Gain=1/MaxEnginePower
  1st Order Reference Model : Subsystem
  AND : Logic  IconShape=distinctive  AllPortsSameDT=off  OutDataTypeStr=boolean
  AND1 : Logic  IconShape=distinctive  AllPortsSameDT=off  OutDataTypeStr=boolean
  Bus Selector1 : BusSelector  OutputSignals=V_mps,hdot_m,Vdot_mps2,altitude_m
  Constant : Constant  Value=ThrottleMax
  Constant1 : Constant  Value=ThrottleMin
  Constant3 : Constant  Value=ThrottleRateMax
  Constant5 : Constant  Value=100
  Divide : Product  Inputs=**
  Gain : Gain  Gain=m/2
  Gain1 : Gain  Gain=m
  Gain2 : Gain  Gain=m*g
  Gain3 : Gain  Gain=m/2
  Gain4 : Gain  Gain=-1
  Gain6 : Gain  Gain=m*g
  Gain7 : Gain  Gain=m*g
  Minus : Sum  Inputs=+-
  NOT : Logic  Operator=NOT  IconShape=distinctive  AllPortsSameDT=off  OutDataTypeStr=boolean
  NOT1 : Logic  Operator=NOT  IconShape=distinctive  AllPortsSameDT=off  OutDataTypeStr=boolean
  NOT2 : Logic  Operator=NOT  IconShape=distinctive  AllPortsSameDT=off  OutDataTypeStr=boolean
  OR : Logic  Operator=OR  IconShape=distinctive  AllPortsSameDT=off  OutDataTypeStr=boolean
  PID Controller : simulink/Continuous/PID Controller  Controller=PID  Form=Parallel  TimeDomain=Discrete-time  SampleTime=dt  IntegratorMethod=Forward Euler  FilterMethod=Forward Euler  ControllerParametersSource=internal  P=PowerError2Throttle  I=PowerErrorInt2Throttle  D=0  UseFilter=on  N=100  TunerSelectOption=Transfer Function Based (PID Tuner App)  InitialConditionSource=internal  InitialConditionForIntegrator=0  InitialConditionForFilter=0  DifferentiatorICPrevScaledInput=0  ExternalReset=level  TrackingMode=off  Kt=1  LimitOutput=off  UpperSaturationLimit=inf  LowerSaturationLimit=-inf  LinearizeAsGain=on  AntiWindupMode=none  Kb=1  POutMin=[]  POutMax=[]  IOutMin=[]  IOutMax=[]  DOutMin=[]  DOutMax=[]  NOutMin=[]  NOutMax=[]  SumOutMin=[]  SumOutMax=[]  SaturationOutMin=[]  SaturationOutMax=[]  PParamMin=[]  PParamMax=[]  IParamMin=[]  IParamMax=[]  DParamMin=[]  DParamMax=[]  NParamMin=[]  NParamMax=[]  KbParamMin=[]  KbParamMax=[]  KtParamMin=[]  KtParamMax=[]  KbOutMin=[]  KbOutMax=[]  KtOutMin=[]  KtOutMax=[]  IntegratorOutMin=[]  IntegratorOutMax=[]  FilterOutMin=[]  FilterOutMax=[]  SumI1OutMin=[]  SumI1OutMax=[]  SumI2OutMin=[]  SumI2OutMax=[]  SumI3OutMin=[]  SumI3OutMax=[]  SumI4OutMin=[]  SumI4OutMax=[]  SumDOutMin=[]  SumDOutMax=[]  DifferentiatorOutMin=[]  DifferentiatorOutMax=[]  FilterDiffOutCoefMin=[]  FilterDiffOutCoefMax=[]  ReciprocalOutMin=[]  ReciprocalOutMax=[]  SumDenOutMin=[]  SumDenOutMax=[]  SumNumOutMin=[]  SumNumOutMax=[]  DivideOutMin=[]  DivideOutMax=[]  IntegratorContinuousStateAttributes=''  IntegratorStateMustResolveToSignalObject=off  IntegratorRTWStateStorageClass=Auto  FilterContinuousStateAttributes=''  FilterStateMustResolveToSignalObject=off  FilterRTWStateStorageClass=Auto  ParallelPVariant=InternalParameters  IdealPVariant=Disabled  IVariant=InternalParameters  DVariant=InternalParameters  IntegratorVariant=Discrete  SatVariant=Disabled  AWVariant=Passthrough  PCopyVariant=Disabled  TRVariant=Disabled  FdbkBlocksVariant=Forward  IdealPFdbkVariant=Disabled  SatFdbkVariant=Disabled  DerivativeFilterVariant=ForwardEulerFilter  NVariant=InternalParameters  NCopyVariant=Disabled  FilterICVariant=InternalICsFilter  IntegratorICVariant=InternalICs  ExternalResetVariant=ExternalReset  TRSumVariant=Passthrough  SumFdbkVariant=Disabled  SumVariant=Sum_PID
  Rate Limiter Dynamic : simulink/Discontinuities/Rate Limiter Dynamic
      settings: SourceProductName=Simulink
  "Saturation " : Saturate  UpperLimit=ThrottleMax  LowerLimit=ThrottleMin  LinearizeAsGain=off
  Square : Math  Operator=square  SaturateOnIntegerOverflow=on
  Square1 : Math  Operator=square  SaturateOnIntegerOverflow=on
  Subsystem : Subsystem
  Sum : Sum  Inputs=|+-
  Sum1 : Sum  Inputs=++|
  Sum4 : Sum  Inputs=|++
  Sum5 : Sum  Inputs=|++
  Sum6 : Sum  Inputs=|++
  Switch{,1..3} (4 alike) : Switch  Criteria=u2 > Threshold  Threshold=0.5
  Throttle (Airspeed TEC) : Outport
  tag scope: AltErr=global, ThrottleCmd=global
  wires:
  Rate Limiter Dynamic/1 -> "Saturation "/1
  Vcmd/1 -> Square/1
  Square/1 -> Gain/1
  Divide/1 -> Gain1/1
  Gain1/1 -> Sum6/2
  Sum/1 -> "1/ MaxEnginePower "/1
  "1/ MaxEnginePower "/1 -> PID Controller/1  "Power Error"
  hCmd/1 -> Gain2/1, Minus/1
  Gain2/1 -> Sum4/1
  1st Order Reference Model/1(Rf) -> Sum/1
  Gain/1 -> 1st Order Reference Model/2(Vcmd), Sum4/2
  Square1/1 -> Gain3/1
  Gain3/1 -> Sum5/1
  Subsystem/1(Throttle Out) -> Switch1/3
  Bus Selector1/3 -> Divide/2  "<Vdot_mps2>"
  " "/1 -> Sum1/1
  "Saturation "/1 -> Throttle (Airspeed TEC)/1, [ThrottleCmd]  "Sim.Throttle (Airspeed)"
  Bus Selector1/1 -> Square1/1, Divide/1, 1st Order Reference Model/4("V ")  "<V_mps>"
  Bus Selector1/2 -> Gain7/1  "<hdot_m>"
  Feedback Bus/1 -> Bus Selector1/1
  Sum4/1 -> 1st Order Reference Model/1(Pcmd)
  Gain6/1 -> Sum5/2
  Sum5/1 -> 1st Order Reference Model/3(Pact)
  Gain7/1 -> Sum6/1
  Sum6/1 -> Sum/2
  Bus Selector1/4 -> Minus/2, Gain6/1  "<altitude_m>"
  Minus/1 -> [AltErr]
  " TLASaturation 1"/1 -> Subsystem/1(Throttle In)
  NOT1/1 -> Subsystem/2(Reset LPF)
  Switch2/1 -> Gain4/1, Rate Limiter Dynamic/1
  [pilotThr] -> Switch/3
  Constant3/1 -> Switch2/1
  Gain4/1 -> Rate Limiter Dynamic/3
  Switch/1 -> " TLASaturation 1"/1
  Constant5/1 -> Switch2/3
  [ApGlobal] -> Switch2/2, Switch/2, NOT1/1, NOT/1
  PID Controller/1 -> Sum1/2
  Sum1/1 -> Switch/1
  NOT/1 -> OR/1
  OR/1 -> PID Controller/2
  NOT2/1 -> OR/2
  [Flag_TAS_Priority] -> NOT2/1
  [Flag_Underspeed] -> AND/1
  [ApGlobal] -> AND/2
  AND/1 -> Switch1/2
  Switch1/1 -> Switch3/3
  Constant/1 -> Switch1/1
  Switch3/1 -> Rate Limiter Dynamic/2
  AND1/1 -> Switch3/2
  [Flag_Overspeed] -> AND1/1
  [ApGlobal] -> AND1/2
  Constant1/1 -> Switch3/1

== system Lib_Piccolo/Throttle Control (Alt Mode) ==
  note: !!!!!!!There is a missing feedforward based on "load factor". This relates to current turn
  hdotCmd : Inport
  TAScmd : Inport  Port=2
  Feedback Bus : Inport  Port=3
  " " : Constant  Value=ThrottleTrim
  " TLASaturation " : Saturate  UpperLimit=ThrottleMax  LowerLimit=ThrottleMin  LinearizeAsGain=off
  "1/ MaxEnginePower " : Gain  Gain=1/MaxEnginePower
  "1/ MaxEnginePower " : Gain  Gain=1/MaxEnginePower
  1st Order Reference Model : Subsystem
  Bus Selector : BusSelector  OutputSignals=V_mps,Vdot_mps2,apMode
  Compare To Constant3 : simulink/Logic and Bit Operations/Compare To Constant  relop=>=  const=11  OutDataTypeStr=boolean
  Constant2 : Constant  Value=0
  Constant3 : Constant  Value=ThrottleRateMax
  Constant4 : Constant  Value=ThrottleControlAltitudeModeIntegratorInit
  Constant5 : Constant  Value=100
  Discrete-Time Integrator1 : DiscreteIntegrator  IntegratorMethod=Integration: Backward Euler  ExternalReset=level  InitialConditionSource=external  SampleTime=-1  LimitOutput=on  UpperSaturationLimit=ThrottleMax-ThrottleTrim  LowerSaturationLimit=ThrottleMin-ThrottleTrim  ICPrevOutput=DiscIntNeverNeededParam  ICPrevScaledInput=DiscIntNeverNeededParam
  Divide : Product  Inputs=**
  EngineKill : Constant  Value=0
  Filter and Throttle Cut : Subsystem
  Flare Throttle Modifications 2 : Subsystem
  Gain : Gain  Gain=m/2
  Gain1 : Gain  Gain=m
  Gain2 : Gain  Gain=m*g
  Gain3 : Gain  Gain=m/2
  Gain4 : Gain  Gain=-1
  KI_Power : Gain  Gain=PowerErrorInt2Throttle
  Kp_Power : Gain  Gain=PowerError2Throttle
  LPF Energy Alpha : Subsystem
  NOT1 : Logic  Operator=NOT  IconShape=distinctive  AllPortsSameDT=off  OutDataTypeStr=boolean
  O/L Throttle Ramp : Subsystem
  Rate Limiter Dynamic : simulink/Discontinuities/Rate Limiter Dynamic
      settings: SourceProductName=Simulink
  Reset Conditions : Subsystem
  Speed Flags : Subsystem
  Square : Math  Operator=square  SaturateOnIntegerOverflow=on
  Square1 : Math  Operator=square  SaturateOnIntegerOverflow=on
  Sum : Sum  Inputs=|+-
  Sum1 : Sum  Inputs=|++
  Sum3 : Sum  Inputs=|++
  Sum4 : Sum  Inputs=+++
  Sum5 : Sum  Inputs=|+-
  Switch : Switch  Criteria=u2 > Threshold  Threshold=0.5
  Switch1 : Switch  Criteria=u2 > Threshold  Threshold=5
  Switch2 : Switch  Criteria=u2 > Threshold  Threshold=0.5
  Switch3 : Switch  Criteria=u2 > Threshold  Threshold=3
  Switch9 : Switch  Criteria=u2 > Threshold
  ThrottlePredictionTrust : Gain  Gain=ThrottlePredictionTrust
  Throttle (Alt TEC) : Outport
  tag scope: Flag_Overspeed=global, Flag_Underspeed=global, Sim_TASError=global, Throttle_Post_Slew=global, Throttle_Pre_Slew=global
  wires:
  TAScmd/1 -> Sum5/1, Switch9/3
  Square/1 -> Gain/1
  Divide/1 -> Gain1/1
  Sum/1 -> "1/ MaxEnginePower "/1
  "1/ MaxEnginePower "/1 -> Kp_Power/1, KI_Power/1  "Sim.Power Error"
  Sum1/1 -> ThrottlePredictionTrust/1
  "1/ MaxEnginePower "/1 -> Sum4/1  "Feedforward_Power"
  1st Order Reference Model/1(Rf) -> Sum1/2, Sum/1
  Gain/1 -> 1st Order Reference Model/1(Pcmd)
  Square1/1 -> Gain3/1
  Bus Selector/2 -> Divide/2  "<Vdot_mps2>"
  Sum5/1 -> [Sim_TASError]  "Sim_TASError"
  LPF Energy Alpha/1(Output) -> Gain2/1
  hdotCmd/1 -> LPF Energy Alpha/1(Input)
  KI_Power/1 -> Discrete-Time Integrator1/1
  Sum4/1 -> Sum3/1  "PI"
  Constant4/1 -> Switch1/1
  Discrete-Time Integrator1/1 -> Sum4/3  "KI_Power"
  Bus Selector/3 -> Reset Conditions/1(AP Mode), Switch3/2, Flare Throttle Modifications 2/3(AP Mode (0 - 12)), Filter and Throttle Cut/3(apMode), Switch1/2, Compare To Constant3/1  "<apMode>"
  ThrottlePredictionTrust/1 -> "1/ MaxEnginePower "/1
  Gain2/1 -> Sum1/1
  Gain3/1 -> 1st Order Reference Model/2(Pact)
  Kp_Power/1 -> Sum4/2  "Kp_Power"
  Switch1/1 -> Discrete-Time Integrator1/3
  Constant2/1 -> Switch9/1
  Gain1/1 -> Sum/2
  Switch9/1 -> Square/1
  Rate Limiter Dynamic/1 -> " TLASaturation "/1
  Sum3/1 -> Switch/1
  Bus Selector/1 -> Sum5/2, Square1/1, 1st Order Reference Model/3("V "), Divide/1  "<V_mps>"
  Compare To Constant3/1 -> Switch9/2
  [ApGlobal] -> Switch/2, Switch2/2, NOT1/1
  NOT1/1 -> Filter and Throttle Cut/2(Reset LPF)
  " TLASaturation "/1 -> Filter and Throttle Cut/1(Throttle In)
  Constant3/1 -> Switch2/1
  Switch2/1 -> Gain4/1, Rate Limiter Dynamic/1
  Gain4/1 -> Rate Limiter Dynamic/3
  Constant5/1 -> Switch2/3
  [pilotThr] -> Switch/3
  Switch/1 -> Rate Limiter Dynamic/2
  " "/1 -> Sum3/2
  Speed Flags/1(Flag_Underspeed) -> [Flag_Underspeed]
  Speed Flags/2(Flag_Overspeed) -> [Flag_Overspeed]
  Filter and Throttle Cut/1(Throttle Out) -> [Throttle_Pre_Slew], Flare Throttle Modifications 2/1(Throttle In (0 - 100%))
  Flare Throttle Modifications 2/1(Throttle Out) -> [Throttle_Post_Slew], Switch3/1
  [PicElevatorOut] -> Flare Throttle Modifications 2/2(Piccolo Elevator In (deg.))
  O/L Throttle Ramp/1(Sim.LaunchThrottleCmd) -> Switch3/3, Switch1/3, Filter and Throttle Cut/4(Throttle Ramp In)
  Feedback Bus/1 -> Bus Selector/1, Speed Flags/1(Feedback Bus), O/L Throttle Ramp/1(Feedback Bus)
  Switch3/1 -> Throttle (Alt TEC)/1
  [startTaxi] -> O/L Throttle Ramp/2(startFlag)
  Reset Conditions/1(Reset) -> Discrete-Time Integrator1/2
  [TakeoffAbortFlag] -> Flare Throttle Modifications 2/5(RTOActive In)
  [ApGlobal] -> Flare Throttle Modifications 2/4(ApGlobal In)
  EngineKill/1 -> Flare Throttle Modifications 2/6(EngineKill In)

== system Lib_Piccolo/VRate Reference Selection ==
  note: Allows Rate Limiter to track current value during AP-off where rates can be arbitrary.
      | Should investigate using a resettable rate limiter to avoid hardcoded value (gross!)
  VRateCmd (Alt) : Inport
  LonMode : Inport  Port=2
  VRateCmd (TAS) : Inport  Port=3
  AND : Logic  IconShape=distinctive  AllPortsSameDT=off  OutDataTypeStr=boolean
  AND1 : Logic  IconShape=distinctive  AllPortsSameDT=off  OutDataTypeStr=boolean
  AND2 : Logic  IconShape=distinctive  AllPortsSameDT=off  OutDataTypeStr=boolean
  Alt Max Accel Rate Limit : Subsystem
  Compare To Constant : simulink/Logic and Bit Operations/Compare To Constant  relop===  const=1  OutDataTypeStr=boolean
  Compare To Constant1 : simulink/Logic and Bit Operations/Compare To Constant  relop=<  const=10  OutDataTypeStr=boolean
  Compare To Constant2 : simulink/Logic and Bit Operations/Compare To Constant  relop=>  const=0  OutDataTypeStr=boolean
  Constant : Constant  Value=Enable_TAS_Protection
  Constant4 : Constant  Value=AltMaxAccel
  Constant5 : Constant  Value=100
  Gain : Gain  Gain=-1
  OR : Logic  Operator=OR  IconShape=distinctive  AllPortsSameDT=off  OutDataTypeStr=boolean
  OR1 : Logic  Operator=OR  IconShape=distinctive  AllPortsSameDT=off  OutDataTypeStr=boolean
  Switch : Switch  Criteria=u2 > Threshold
  Switch2 : Switch  Criteria=u2 > Threshold  Threshold=0.5
  VRateCmd : Outport
  tag scope: Flag_TAS_Priority=global
  wires:
  Switch/1 -> Alt Max Accel Rate Limit/2(u)
  Alt Max Accel Rate Limit/1(Y) -> VRateCmd/1  "Sim.VRateCmd"
  Compare To Constant/1 -> OR/1
  LonMode/1 -> Compare To Constant/1
  VRateCmd (Alt)/1 -> Switch/3
  VRateCmd (TAS)/1 -> Switch/1
  AND/1 -> AND1/1, Switch/2  "Flag_TAS_Priority"
  Constant5/1 -> Switch2/3
  Switch2/1 -> Alt Max Accel Rate Limit/1(up), Gain/1  "altAccelLimit"
  [ApGlobal] -> Switch2/2
  Constant4/1 -> Switch2/1
  Gain/1 -> Alt Max Accel Rate Limit/3(lo)
  [ApGlobal] -> AND/1
  OR/1 -> AND/2
  AND1/1 -> [Flag_TAS_Priority]
  Compare To Constant1/1 -> AND1/2
  [Pic_AP_Mode] -> Compare To Constant1/1
  Compare To Constant2/1 -> AND2/2
  Constant/1 -> Compare To Constant2/1
  [Flag_Underspeed] -> OR1/1
  [Flag_Overspeed] -> OR1/2
  OR1/1 -> AND2/1
  AND2/1 -> OR/2
